simulink model "fw_sbus_decoder"  (R2026b)
settings: Solver=VariableStepAuto
undefined symbols (not defined in the file or in its folder): P, Ts
libraries: simulink x5
settings Model: Creator=aomar  LastModifiedBy=aomar

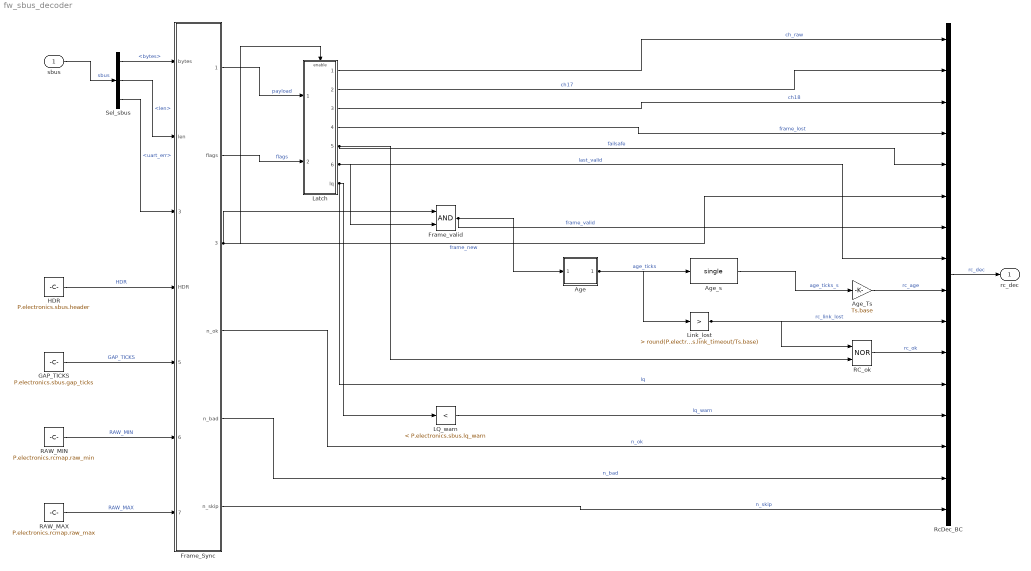
== system fw_sbus_decoder ==
  sbus : Inport  OutDataTypeStr=Bus: Bus_SbusStream  SampleTime=Ts.base
  Age : Subsystem
  Age_Ts : Gain  Gain=Ts.base
  Age_s : DataTypeConversion  OutDataTypeStr=single  RndMeth=Round
  Frame_Sync : MATLAB Function  TreatAsAtomicUnit=on
  Frame_valid : Logic  AllPortsSameDT=off  OutDataTypeStr=boolean
  GAP_TICKS : Constant  Value=P.electronics.sbus.gap_ticks  OutDataTypeStr=uint8  SampleTime=Ts.base
  HDR : Constant  Value=P.electronics.sbus.header  OutDataTypeStr=uint8  SampleTime=Ts.base
  LQ_warn : simulink/Logic and Bit Operations/Compare To Constant  relop=<  const=P.electronics.sbus.lq_warn  OutDataTypeStr=boolean
  Latch : Subsystem
  Link_lost : simulink/Logic and Bit Operations/Compare To Constant  relop=>  const=round(P.electronics.sbus.link_timeout/Ts.base)  OutDataTypeStr=boolean
  RAW_MAX : Constant  Value=P.electronics.rcmap.raw_max  OutDataTypeStr=uint16  SampleTime=Ts.base
  RAW_MIN : Constant  Value=P.electronics.rcmap.raw_min  OutDataTypeStr=uint16  SampleTime=Ts.base
  RC_ok : Logic  Operator=NOR  AllPortsSameDT=off  OutDataTypeStr=boolean
  RcDec_BC : BusCreator  Inputs=16
  Sel_sbus : BusSelector  OutputSignals=bytes,len,uart_err
  rc_dec : Outport
  wires:
  sbus/1 -> Sel_sbus/1  "sbus"
  HDR/1 -> Frame_Sync/4(HDR)  "HDR"
  GAP_TICKS/1 -> Frame_Sync/5(GAP_TICKS)  "GAP_TICKS"
  RAW_MIN/1 -> Frame_Sync/6(RAW_MIN)  "RAW_MIN"
  RAW_MAX/1 -> Frame_Sync/7(RAW_MAX)  "RAW_MAX"
  Sel_sbus/1 -> Frame_Sync/1(bytes)  "<bytes>"
  Sel_sbus/2 -> Frame_Sync/2(len)  "<len>"
  Sel_sbus/3 -> Frame_Sync/3(uart_err)  "<uart_err>"
  Frame_Sync/1(payload) -> Latch/1(payload)  "payload"
  Frame_Sync/2(flags) -> Latch/2(flags)  "flags"
  Frame_Sync/3(frame_new) -> Latch/Enable, RcDec_BC/6, Frame_valid/1  "frame_new"
  Frame_Sync/4(n_ok) -> RcDec_BC/14  "n_ok"
  Frame_Sync/5(n_bad) -> RcDec_BC/15  "n_bad"
  Frame_Sync/6(n_skip) -> RcDec_BC/16  "n_skip"
  Latch/1(ch_raw) -> RcDec_BC/1  "ch_raw"
  Latch/2(ch17) -> RcDec_BC/2  "ch17"
  Latch/3(ch18) -> RcDec_BC/3  "ch18"
  Latch/4(frame_lost) -> RcDec_BC/4  "frame_lost"
  Frame_valid/1 -> Age/1(fresh), RcDec_BC/7  "frame_valid"
  LQ_warn/1 -> RcDec_BC/13  "lq_warn"
  Age/1(ticks) -> Link_lost/1, Age_s/1  "age_ticks"
  Link_lost/1 -> RC_ok/1, RcDec_BC/10  "rc_link_lost"
  Age_s/1 -> Age_Ts/1  "age_ticks_s"
  Age_Ts/1 -> RcDec_BC/9  "rc_age"
  RC_ok/1 -> RcDec_BC/11  "rc_ok"
  RcDec_BC/1 -> rc_dec/1  "rc_dec"
  Latch/6(last_valid) -> RcDec_BC/8, Frame_valid/2  "last_valid"
  Latch/7(lq) -> LQ_warn/1, RcDec_BC/12  "lq"
  Latch/5(failsafe) -> RC_ok/2, RcDec_BC/5  "failsafe"

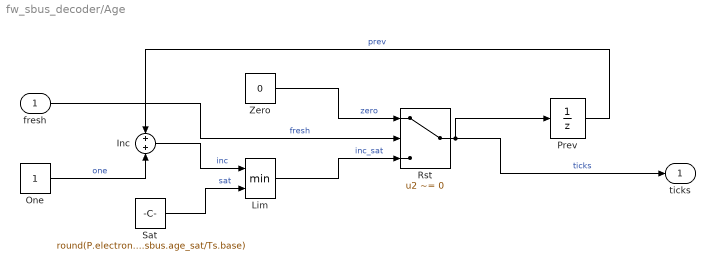
== system fw_sbus_decoder/Age ==
  fresh : Inport
  Inc : Sum  OutDataTypeStr=uint16  SaturateOnIntegerOverflow=on
  Lim : MinMax  Inputs=2
  One : Constant  OutDataTypeStr=uint16  SampleTime=-1
  Prev : UnitDelay  InitialCondition=round(P.electronics.sbus.age_sat/Ts.base)  SampleTime=-1
  Rst : Switch  Criteria=u2 ~= 0  SaturateOnIntegerOverflow=off  InputSameDT=off
  Sat : Constant  Value=round(P.electronics.sbus.age_sat/Ts.base)  OutDataTypeStr=uint16  SampleTime=-1
  Zero : Constant  Value=0  OutDataTypeStr=uint16  SampleTime=-1
  ticks : Outport
  wires:
  fresh/1 -> Rst/2  "fresh"
  One/1 -> Inc/2  "one"
  Inc/1 -> Lim/1  "inc"
  Sat/1 -> Lim/2  "sat"
  Zero/1 -> Rst/1  "zero"
  Lim/1 -> Rst/3  "inc_sat"
  Rst/1 -> ticks/1, Prev/1  "ticks"
  Prev/1 -> Inc/1  "prev"

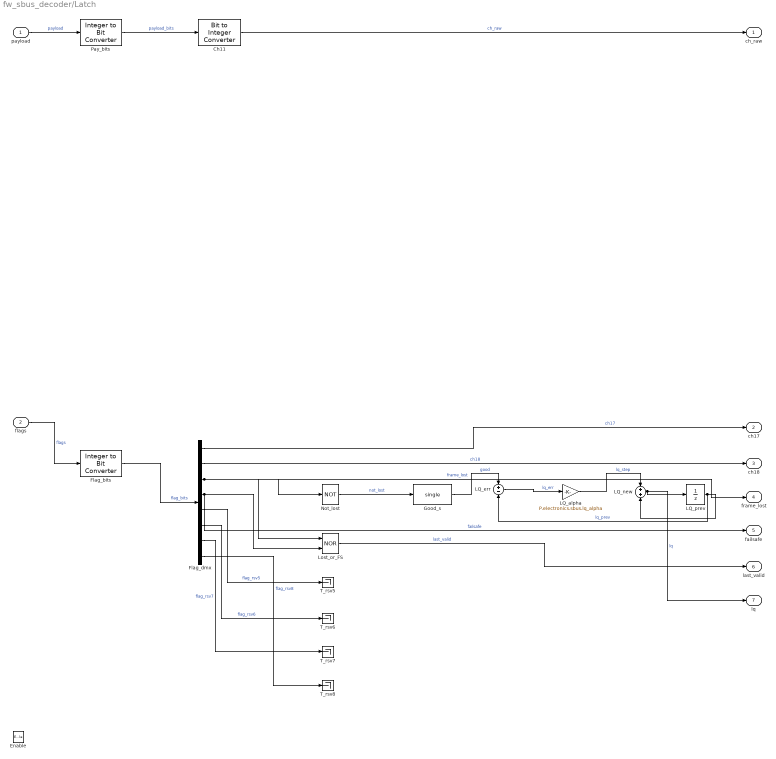
== system fw_sbus_decoder/Latch ==
  payload : Inport
  flags : Inport  Port=2
  Enable : EnablePort
  Ch11 : simulink/Logic and Bit Operations/Bit to Integer Converter  nbits=P.electronics.sbus.ch_bits  bitOrder=LSB first  signedOutputValues=Unsigned  outDtype=uint16  outDtypeSigned=Inherit via internal rule
      settings: LibrarySourceBlock=|
      | commutil2/Bit to Integer
      | Converter
  Flag_bits : simulink/Logic and Bit Operations/Integer to Bit Converter  nbits=8  signedInputValues=Unsigned  bitOrder=LSB first  outDtype=boolean
      settings: LibrarySourceBlock=|
      | commutil2/Integer to Bit
      | Converter
  Flag_dmx : Demux  Outputs=8
  Good_s : DataTypeConversion  OutDataTypeStr=single  RndMeth=Round
  LQ_alpha : Gain  Gain=P.electronics.sbus.lq_alpha
  LQ_err : Sum  Inputs=+-
  LQ_new : Sum
  LQ_prev : UnitDelay  InitialCondition=single(P.electronics.sbus.lq_ic)  SampleTime=-1
  Lost_or_FS : Logic  Operator=NOR  AllPortsSameDT=off  OutDataTypeStr=boolean
  Not_lost : Logic  Operator=NOT  Inputs=1  AllPortsSameDT=off  OutDataTypeStr=boolean
  Pay_bits : simulink/Logic and Bit Operations/Integer to Bit Converter  nbits=8  signedInputValues=Unsigned  bitOrder=LSB first  outDtype=boolean
      settings: LibrarySourceBlock=|
      | commutil2/Integer to Bit
      | Converter
  T_rsv{5..8} (4 alike) : Terminator
  ch_raw : Outport  InitialOutput=uint16(P.electronics.rcmap.raw_mid)
  ch17 : Outport  Port=2  InitialOutput=false
  ch18 : Outport  Port=3  InitialOutput=false
  frame_lost : Outport  Port=4  InitialOutput=false
  failsafe : Outport  Port=5  InitialOutput=false
  last_valid : Outport  Port=6  InitialOutput=false
  lq : Outport  Port=7  InitialOutput=single(P.electronics.sbus.lq_ic)
  wires:
  payload/1 -> Pay_bits/1  "payload"
  flags/1 -> Flag_bits/1  "flags"
  Pay_bits/1 -> Ch11/1  "payload_bits"
  Flag_bits/1 -> Flag_dmx/1  "flag_bits"
  Flag_dmx/1 -> ch17/1  "ch17"
  Flag_dmx/2 -> ch18/1  "ch18"
  Flag_dmx/5 -> T_rsv5/1  "flag_rsv5"
  Flag_dmx/6 -> T_rsv6/1  "flag_rsv6"
  Flag_dmx/7 -> T_rsv7/1  "flag_rsv7"
  Flag_dmx/8 -> T_rsv8/1  "flag_rsv8"
  Ch11/1 -> ch_raw/1  "ch_raw"
  Not_lost/1 -> Good_s/1  "not_lost"
  Lost_or_FS/1 -> last_valid/1  "last_valid"
  Good_s/1 -> LQ_err/1  "good"
  LQ_err/1 -> LQ_alpha/1  "lq_err"
  LQ_alpha/1 -> LQ_new/1  "lq_step"
  LQ_new/1 -> lq/1, LQ_prev/1  "lq"
  LQ_prev/1 -> LQ_new/2, LQ_err/2  "lq_prev"
  Flag_dmx/3 -> Lost_or_FS/1, frame_lost/1, Not_lost/1  "frame_lost"
  Flag_dmx/4 -> Lost_or_FS/2, failsafe/1  "failsafe"

== matlab function fw_sbus_decoder/Frame_Sync ==
  settings: description=SBUS frame synchroniser (spec 4.1, rev. C: a UART error taints every frame with a byte in the flagged chunk; 25-byte length, footer, reserved flag bits, channel range RAW_MIN..RAW_MAX). HDR / GAP_TICKS / RAW_MIN / RAW_MAX arrive on inputs (no parameter data).
  data: bytes input; payload output; len input; uart_err input; HDR input; GAP_TICKS input; RAW_MIN input; RAW_MAX input; flags output; frame_new output; n_ok output; n_bad output; n_skip output
function [payload, flags, frame_new, n_ok, n_bad, n_skip] = fcn(bytes, len, uart_err, HDR, GAP_TICKS, RAW_MIN, RAW_MAX)
%#codegen
% body: subsystems/electronics/sbus_frame_sync.m (docs/specs/electronics.md 4.1, revision C)
[payload, flags, frame_new, n_ok, n_bad, n_skip] = sbus_frame_sync(bytes, len, uart_err, HDR, GAP_TICKS, RAW_MIN, RAW_MAX);
